simulink library "xps_library"  (Simulink 8.0)
settings: Solver=ode45  SolverMode=SingleTasking  StartTime=0.0  StopTime=10.0  RelTol=1e-3
undefined symbols (not defined in the file): sys_clk, xps_library_software_register_user_data_in
libraries: xbsIndex_r4 x867, simulink x109, dspsigops x81, casper_library_flow_control x68, xps_library x18, casper_library_misc x11
(part 5 of 10)

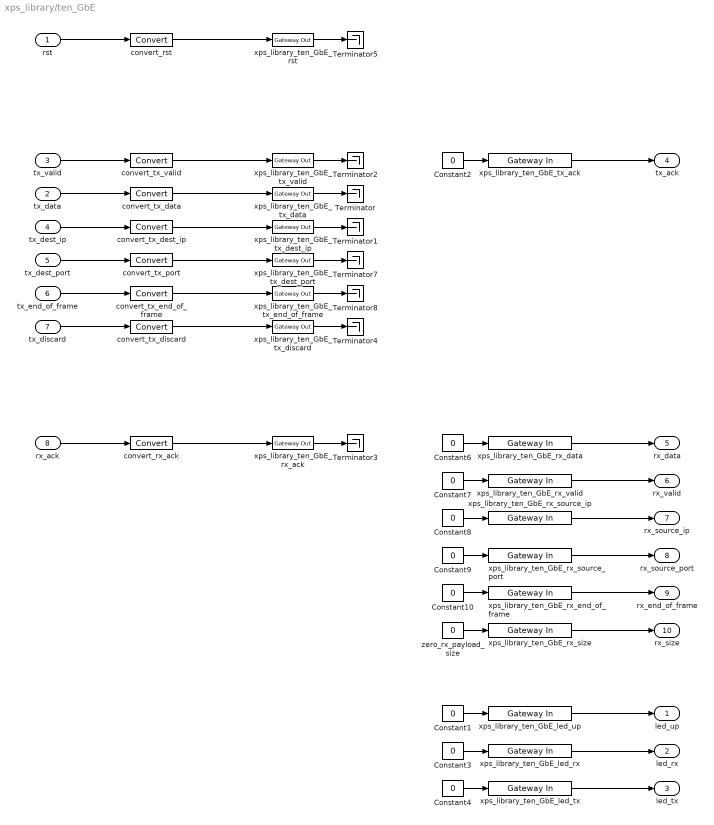
== system xps_library/ten_GbE ==
  rst : Inport
  tx_data : Inport  Port=2
  tx_valid : Inport  Port=3
  tx_dest_ip : Inport  Port=4
  tx_dest_port : Inport  Port=5
  tx_end_of_frame : Inport  Port=6
  tx_discard : Inport  Port=7
  rx_ack : Inport  Port=8
  Constant{1..4,6..10} (9 alike) : Constant  Value=0
  Terminator{,1..5,7..8} (8 alike) : Terminator
  convert_rst : xbsIndex_r4/Convert  gui_display_data_type=Fixed-point  arith_type=Boolean  n_bits=64  bin_pt=0  float_type=Single  exp_bits=8  fraction_bits=24  quantization=Truncate  overflow=Wrap  en=off  latency=0  dbl_ovrd=off  pipeline=off  block_type=convert
      settings: xl_area=[0, 0, 0, 0, 0, 0, 0]
  convert_rx_ack : xbsIndex_r4/Convert  gui_display_data_type=Fixed-point  arith_type=Boolean  n_bits=64  bin_pt=0  float_type=Single  exp_bits=8  fraction_bits=24  quantization=Truncate  overflow=Wrap  en=off  latency=0  dbl_ovrd=off  pipeline=off  block_type=convert
      settings: xl_area=[0, 0, 0, 0, 0, 0, 0]
  convert_tx_data : xbsIndex_r4/Convert  gui_display_data_type=Fixed-point  arith_type=Unsigned  n_bits=64  bin_pt=0  float_type=Single  exp_bits=8  fraction_bits=24  quantization=Truncate  overflow=Wrap  en=off  latency=0  dbl_ovrd=off  pipeline=off  block_type=convert
      settings: xl_area=[0, 0, 0, 0, 0, 0, 0]
  convert_tx_dest_ip : xbsIndex_r4/Convert  gui_display_data_type=Fixed-point  arith_type=Unsigned  n_bits=32  bin_pt=0  float_type=Single  exp_bits=8  fraction_bits=24  quantization=Truncate  overflow=Wrap  en=off  latency=0  dbl_ovrd=off  pipeline=off  block_type=convert
      settings: xl_area=[0, 0, 0, 0, 0, 0, 0]
  convert_tx_discard : xbsIndex_r4/Convert  gui_display_data_type=Fixed-point  arith_type=Boolean  n_bits=1  bin_pt=0  float_type=Single  exp_bits=8  fraction_bits=24  quantization=Truncate  overflow=Wrap  en=off  latency=0  dbl_ovrd=off  pipeline=off  block_type=convert
      settings: xl_area=[0, 0, 0, 0, 0, 0, 0]
  convert_tx_end_of_frame : xbsIndex_r4/Convert  gui_display_data_type=Fixed-point  arith_type=Boolean  n_bits=1  bin_pt=0  float_type=Single  exp_bits=8  fraction_bits=24  quantization=Truncate  overflow=Wrap  en=off  latency=0  dbl_ovrd=off  pipeline=off  block_type=convert
      settings: xl_area=[0, 0, 0, 0, 0, 0, 0]
  convert_tx_port : xbsIndex_r4/Convert  gui_display_data_type=Fixed-point  arith_type=Unsigned  n_bits=16  bin_pt=0  float_type=Single  exp_bits=8  fraction_bits=24  quantization=Truncate  overflow=Wrap  en=off  latency=0  dbl_ovrd=off  pipeline=off  block_type=convert
      settings: xl_area=[0, 0, 0, 0, 0, 0, 0]
  convert_tx_valid : xbsIndex_r4/Convert  gui_display_data_type=Fixed-point  arith_type=Boolean  n_bits=1  bin_pt=0  float_type=Single  exp_bits=8  fraction_bits=24  quantization=Truncate  overflow=Wrap  en=off  latency=0  dbl_ovrd=off  pipeline=off  block_type=convert
      settings: xl_area=[0, 0, 0, 0, 0, 0, 0]
  xps_library_ten_GbE_led_rx : xbsIndex_r4/Gateway In  gui_display_data_type=Fixed-point  arith_type=Boolean  n_bits=1  bin_pt=0  preci_type=Single  exp_width=8  frac_width=24  quantization=Truncate  overflow=Wrap  period=1  dbl_ovrd=off  timing_constraint=None  locs_specified=off  LOCs={}  hdl_port=on  block_type=gatewayin
      settings: infoedit="Gateway in block.  Converts inputs of type Simulink integer, double and fixed point to  Xilinx fixed point type.<P><P>Hardware notes:  In hardware these blocks become top level input ports."  xl_area=[0, 0, 0, 0, 0, 0, 0]
  xps_library_ten_GbE_led_tx : xbsIndex_r4/Gateway In  gui_display_data_type=Fixed-point  arith_type=Boolean  n_bits=1  bin_pt=0  preci_type=Single  exp_width=8  frac_width=24  quantization=Truncate  overflow=Wrap  period=1  dbl_ovrd=off  timing_constraint=None  locs_specified=off  LOCs={}  hdl_port=on  block_type=gatewayin
      settings: infoedit="Gateway in block.  Converts inputs of type Simulink integer, double and fixed point to  Xilinx fixed point type.<P><P>Hardware notes:  In hardware these blocks become top level input ports."  xl_area=[0, 0, 0, 0, 0, 0, 0]
  xps_library_ten_GbE_led_up : xbsIndex_r4/Gateway In  gui_display_data_type=Fixed-point  arith_type=Boolean  n_bits=1  bin_pt=0  preci_type=Single  exp_width=8  frac_width=24  quantization=Truncate  overflow=Wrap  period=1  dbl_ovrd=off  timing_constraint=None  locs_specified=off  LOCs={}  hdl_port=on  block_type=gatewayin
      settings: infoedit="Gateway in block.  Converts inputs of type Simulink integer, double and fixed point to  Xilinx fixed point type.<P><P>Hardware notes:  In hardware these blocks become top level input ports."  xl_area=[0, 0, 0, 0, 0, 0, 0]
  xps_library_ten_GbE_rst : xbsIndex_r4/Gateway Out  hdl_port=on  timing_constraint=None  locs_specified=off  LOCs={}  block_type=gatewayout
      settings: infoedit="Gateway out block.  Converts Xilinx fixed point inputs into ouputs of type Simulink integer, double, or fixed point.<P><P>Hardware notes:  In hardware these blocks become top level output ports or are discarded, depending on how they are configured."  xl_area=[0, 0, 0, 0, 0, 0, 0]
  xps_library_ten_GbE_rx_ack : xbsIndex_r4/Gateway Out  hdl_port=on  timing_constraint=None  locs_specified=off  LOCs={}  block_type=gatewayout
      settings: infoedit="Gateway out block.  Converts Xilinx fixed point inputs into ouputs of type Simulink integer, double, or fixed point.<P><P>Hardware notes:  In hardware these blocks become top level output ports or are discarded, depending on how they are configured."  xl_area=[0, 0, 0, 0, 0, 0, 0]
  xps_library_ten_GbE_rx_data : xbsIndex_r4/Gateway In  gui_display_data_type=Fixed-point  arith_type=Unsigned  n_bits=64  bin_pt=0  preci_type=Single  exp_width=8  frac_width=24  quantization=Truncate  overflow=Wrap  period=1  dbl_ovrd=off  timing_constraint=None  locs_specified=off  LOCs={}  hdl_port=on  block_type=gatewayin
      settings: infoedit="Gateway in block.  Converts inputs of type Simulink integer, double and fixed point to  Xilinx fixed point type.<P><P>Hardware notes:  In hardware these blocks become top level input ports."  xl_area=[0, 0, 0, 0, 0, 0, 0]
  xps_library_ten_GbE_rx_end_of_frame : xbsIndex_r4/Gateway In  gui_display_data_type=Fixed-point  arith_type=Boolean  n_bits=1  bin_pt=0  preci_type=Single  exp_width=8  frac_width=24  quantization=Truncate  overflow=Wrap  period=1  dbl_ovrd=off  timing_constraint=None  locs_specified=off  LOCs={}  hdl_port=on  block_type=gatewayin
      settings: infoedit="Gateway in block.  Converts inputs of type Simulink integer, double and fixed point to  Xilinx fixed point type.<P><P>Hardware notes:  In hardware these blocks become top level input ports."  xl_area=[0, 0, 0, 0, 0, 0, 0]
  xps_library_ten_GbE_rx_size : xbsIndex_r4/Gateway In  gui_display_data_type=Fixed-point  arith_type=Unsigned  n_bits=16  bin_pt=0  preci_type=Single  exp_width=8  frac_width=24  quantization=Truncate  overflow=Wrap  period=1  dbl_ovrd=off  timing_constraint=None  locs_specified=off  LOCs={}  hdl_port=on  block_type=gatewayin
      settings: infoedit="Gateway in block.  Converts inputs of type Simulink integer, double and fixed point to  Xilinx fixed point type.<P><P>Hardware notes:  In hardware these blocks become top level input ports."  xl_area=[0, 0, 0, 0, 0, 0, 0]
  xps_library_ten_GbE_rx_source_ip : xbsIndex_r4/Gateway In  gui_display_data_type=Fixed-point  arith_type=Unsigned  n_bits=32  bin_pt=0  preci_type=Single  exp_width=8  frac_width=24  quantization=Truncate  overflow=Wrap  period=1  dbl_ovrd=off  timing_constraint=None  locs_specified=off  LOCs={}  hdl_port=on  block_type=gatewayin
      settings: infoedit="Gateway in block.  Converts inputs of type Simulink integer, double and fixed point to  Xilinx fixed point type.<P><P>Hardware notes:  In hardware these blocks become top level input ports."  xl_area=[0, 0, 0, 0, 0, 0, 0]
  xps_library_ten_GbE_rx_source_port : xbsIndex_r4/Gateway In  gui_display_data_type=Fixed-point  arith_type=Unsigned  n_bits=16  bin_pt=0  preci_type=Single  exp_width=8  frac_width=24  quantization=Truncate  overflow=Wrap  period=1  dbl_ovrd=off  timing_constraint=None  locs_specified=off  LOCs={}  hdl_port=on  block_type=gatewayin
      settings: infoedit="Gateway in block.  Converts inputs of type Simulink integer, double and fixed point to  Xilinx fixed point type.<P><P>Hardware notes:  In hardware these blocks become top level input ports."  xl_area=[0, 0, 0, 0, 0, 0, 0]
  xps_library_ten_GbE_rx_valid : xbsIndex_r4/Gateway In  gui_display_data_type=Fixed-point  arith_type=Boolean  n_bits=1  bin_pt=0  preci_type=Single  exp_width=8  frac_width=24  quantization=Truncate  overflow=Wrap  period=1  dbl_ovrd=off  timing_constraint=None  locs_specified=off  LOCs={}  hdl_port=on  block_type=gatewayin
      settings: infoedit="Gateway in block.  Converts inputs of type Simulink integer, double and fixed point to  Xilinx fixed point type.<P><P>Hardware notes:  In hardware these blocks become top level input ports."  xl_area=[0, 0, 0, 0, 0, 0, 0]
  xps_library_ten_GbE_tx_ack : xbsIndex_r4/Gateway In  gui_display_data_type=Fixed-point  arith_type=Boolean  n_bits=1  bin_pt=0  preci_type=Single  exp_width=8  frac_width=24  quantization=Truncate  overflow=Wrap  period=1  dbl_ovrd=off  timing_constraint=None  locs_specified=off  LOCs={}  hdl_port=on  block_type=gatewayin
      settings: infoedit="Gateway in block.  Converts inputs of type Simulink integer, double and fixed point to  Xilinx fixed point type.<P><P>Hardware notes:  In hardware these blocks become top level input ports."  xl_area=[0, 0, 0, 0, 0, 0, 0]
  xps_library_ten_GbE_tx_data : xbsIndex_r4/Gateway Out  hdl_port=on  timing_constraint=None  locs_specified=off  LOCs={}  block_type=gatewayout
      settings: infoedit="Gateway out block.  Converts Xilinx fixed point inputs into ouputs of type Simulink integer, double, or fixed point.<P><P>Hardware notes:  In hardware these blocks become top level output ports or are discarded, depending on how they are configured."  xl_area=[0, 0, 0, 0, 0, 0, 0]
  xps_library_ten_GbE_tx_dest_ip : xbsIndex_r4/Gateway Out  hdl_port=on  timing_constraint=None  locs_specified=off  LOCs={}  block_type=gatewayout
      settings: infoedit="Gateway out block.  Converts Xilinx fixed point inputs into ouputs of type Simulink integer, double, or fixed point.<P><P>Hardware notes:  In hardware these blocks become top level output ports or are discarded, depending on how they are configured."  xl_area=[0, 0, 0, 0, 0, 0, 0]
  xps_library_ten_GbE_tx_dest_port : xbsIndex_r4/Gateway Out  hdl_port=on  timing_constraint=None  locs_specified=off  LOCs={}  block_type=gatewayout
      settings: infoedit="Gateway out block.  Converts Xilinx fixed point inputs into ouputs of type Simulink integer, double, or fixed point.<P><P>Hardware notes:  In hardware these blocks become top level output ports or are discarded, depending on how they are configured."  xl_area=[0, 0, 0, 0, 0, 0, 0]
  xps_library_ten_GbE_tx_discard : xbsIndex_r4/Gateway Out  hdl_port=on  timing_constraint=None  locs_specified=off  LOCs={}  block_type=gatewayout
      settings: infoedit="Gateway out block.  Converts Xilinx fixed point inputs into ouputs of type Simulink integer, double, or fixed point.<P><P>Hardware notes:  In hardware these blocks become top level output ports or are discarded, depending on how they are configured."  xl_area=[0, 0, 0, 0, 0, 0, 0]
  xps_library_ten_GbE_tx_end_of_frame : xbsIndex_r4/Gateway Out  hdl_port=on  timing_constraint=None  locs_specified=off  LOCs={}  block_type=gatewayout
      settings: infoedit="Gateway out block.  Converts Xilinx fixed point inputs into ouputs of type Simulink integer, double, or fixed point.<P><P>Hardware notes:  In hardware these blocks become top level output ports or are discarded, depending on how they are configured."  xl_area=[0, 0, 0, 0, 0, 0, 0]
  xps_library_ten_GbE_tx_valid : xbsIndex_r4/Gateway Out  hdl_port=on  timing_constraint=None  locs_specified=off  LOCs={}  block_type=gatewayout
      settings: infoedit="Gateway out block.  Converts Xilinx fixed point inputs into ouputs of type Simulink integer, double, or fixed point.<P><P>Hardware notes:  In hardware these blocks become top level output ports or are discarded, depending on how they are configured."  xl_area=[0, 0, 0, 0, 0, 0, 0]
  zero_rx_payload_size : Constant  Value=0
  led_up : Outport
  led_rx : Outport  Port=2
  led_tx : Outport  Port=3
  tx_ack : Outport  Port=4
  rx_data : Outport  Port=5
  rx_valid : Outport  Port=6
  rx_source_ip : Outport  Port=7
  rx_source_port : Outport  Port=8
  rx_end_of_frame : Outport  Port=9
  rx_size : Outport  Port=10
  wires:
  rx_ack/1 -> convert_rx_ack/1
  convert_rx_ack/1 -> xps_library_ten_GbE_rx_ack/1
  xps_library_ten_GbE_rx_data/1 -> rx_data/1
  tx_data/1 -> convert_tx_data/1
  convert_tx_data/1 -> xps_library_ten_GbE_tx_data/1
  tx_dest_ip/1 -> convert_tx_dest_ip/1
  convert_tx_dest_ip/1 -> xps_library_ten_GbE_tx_dest_ip/1
  tx_valid/1 -> convert_tx_valid/1
  convert_tx_valid/1 -> xps_library_ten_GbE_tx_valid/1
  xps_library_ten_GbE_tx_ack/1 -> tx_ack/1
  xps_library_ten_GbE_tx_data/1 -> Terminator/1
  xps_library_ten_GbE_tx_dest_ip/1 -> Terminator1/1
  xps_library_ten_GbE_tx_valid/1 -> Terminator2/1
  Constant2/1 -> xps_library_ten_GbE_tx_ack/1
  Constant6/1 -> xps_library_ten_GbE_rx_data/1
  xps_library_ten_GbE_rx_ack/1 -> Terminator3/1
  Constant7/1 -> xps_library_ten_GbE_rx_valid/1
  xps_library_ten_GbE_rx_valid/1 -> rx_valid/1
  rst/1 -> convert_rst/1
  convert_rst/1 -> xps_library_ten_GbE_rst/1
  xps_library_ten_GbE_rst/1 -> Terminator5/1
  tx_dest_port/1 -> convert_tx_port/1
  convert_tx_port/1 -> xps_library_ten_GbE_tx_dest_port/1
  xps_library_ten_GbE_tx_dest_port/1 -> Terminator7/1
  tx_end_of_frame/1 -> convert_tx_end_of_frame/1
  convert_tx_end_of_frame/1 -> xps_library_ten_GbE_tx_end_of_frame/1
  xps_library_ten_GbE_tx_end_of_frame/1 -> Terminator8/1
  xps_library_ten_GbE_rx_source_ip/1 -> rx_source_ip/1
  Constant8/1 -> xps_library_ten_GbE_rx_source_ip/1
  Constant9/1 -> xps_library_ten_GbE_rx_source_port/1
  xps_library_ten_GbE_rx_source_port/1 -> rx_source_port/1
  Constant10/1 -> xps_library_ten_GbE_rx_end_of_frame/1
  xps_library_ten_GbE_rx_end_of_frame/1 -> rx_end_of_frame/1
  Constant1/1 -> xps_library_ten_GbE_led_up/1
  xps_library_ten_GbE_led_up/1 -> led_up/1
  Constant3/1 -> xps_library_ten_GbE_led_rx/1
  xps_library_ten_GbE_led_rx/1 -> led_rx/1
  Constant4/1 -> xps_library_ten_GbE_led_tx/1
  xps_library_ten_GbE_led_tx/1 -> led_tx/1
  zero_rx_payload_size/1 -> xps_library_ten_GbE_rx_size/1
  xps_library_ten_GbE_rx_size/1 -> rx_size/1
  tx_discard/1 -> convert_tx_discard/1
  convert_tx_discard/1 -> xps_library_ten_GbE_tx_discard/1
  xps_library_ten_GbE_tx_discard/1 -> Terminator4/1

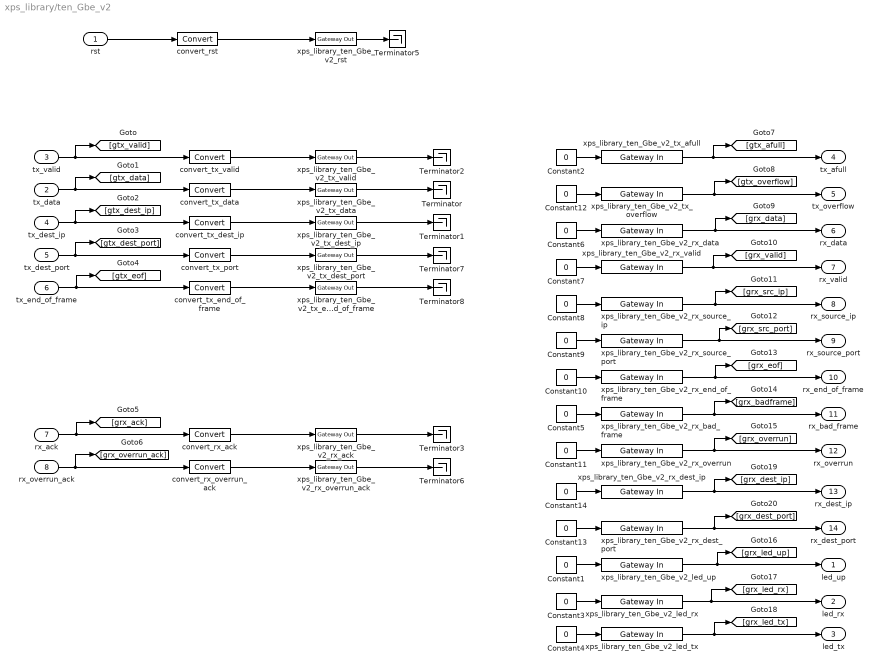
== system xps_library/ten_Gbe_v2 ==
  rst : Inport
  tx_data : Inport  Port=2
  tx_valid : Inport  Port=3
  tx_dest_ip : Inport  Port=4
  tx_dest_port : Inport  Port=5
  tx_end_of_frame : Inport  Port=6
  rx_ack : Inport  Port=7
  rx_overrun_ack : Inport  Port=8
  Constant{1..14} (14 alike) : Constant  Value=0
  Terminator{,1..3,5..8} (8 alike) : Terminator
  convert_rst : xbsIndex_r4/Convert  gui_display_data_type=Fixed-point  arith_type=Boolean  n_bits=64  bin_pt=0  float_type=Single  exp_bits=8  fraction_bits=24  quantization=Truncate  overflow=Wrap  en=off  latency=0  dbl_ovrd=off  pipeline=off  block_type=convert
      settings: xl_area=[0, 0, 0, 0, 0, 0, 0]
  convert_rx_ack : xbsIndex_r4/Convert  gui_display_data_type=Fixed-point  arith_type=Boolean  n_bits=64  bin_pt=0  float_type=Single  exp_bits=8  fraction_bits=24  quantization=Truncate  overflow=Wrap  en=off  latency=0  dbl_ovrd=off  pipeline=off  block_type=convert
      settings: xl_area=[0, 0, 0, 0, 0, 0, 0]
  convert_rx_overrun_ack : xbsIndex_r4/Convert  gui_display_data_type=Fixed-point  arith_type=Boolean  n_bits=64  bin_pt=0  float_type=Single  exp_bits=8  fraction_bits=24  quantization=Truncate  overflow=Wrap  en=off  latency=0  dbl_ovrd=off  pipeline=off  block_type=convert
      settings: xl_area=[0, 0, 0, 0, 0, 0, 0]
  convert_tx_data : xbsIndex_r4/Convert  gui_display_data_type=Fixed-point  arith_type=Unsigned  n_bits=64  bin_pt=0  float_type=Single  exp_bits=8  fraction_bits=24  quantization=Truncate  overflow=Wrap  en=off  latency=0  dbl_ovrd=off  pipeline=off  block_type=convert
      settings: xl_area=[0, 0, 0, 0, 0, 0, 0]
  convert_tx_dest_ip : xbsIndex_r4/Convert  gui_display_data_type=Fixed-point  arith_type=Unsigned  n_bits=32  bin_pt=0  float_type=Single  exp_bits=8  fraction_bits=24  quantization=Truncate  overflow=Wrap  en=off  latency=0  dbl_ovrd=off  pipeline=off  block_type=convert
      settings: xl_area=[0, 0, 0, 0, 0, 0, 0]
  convert_tx_end_of_frame : xbsIndex_r4/Convert  gui_display_data_type=Fixed-point  arith_type=Boolean  n_bits=1  bin_pt=0  float_type=Single  exp_bits=8  fraction_bits=24  quantization=Truncate  overflow=Wrap  en=off  latency=0  dbl_ovrd=off  pipeline=off  block_type=convert
      settings: xl_area=[0, 0, 0, 0, 0, 0, 0]
  convert_tx_port : xbsIndex_r4/Convert  gui_display_data_type=Fixed-point  arith_type=Unsigned  n_bits=16  bin_pt=0  float_type=Single  exp_bits=8  fraction_bits=24  quantization=Truncate  overflow=Wrap  en=off  latency=0  dbl_ovrd=off  pipeline=off  block_type=convert
      settings: xl_area=[0, 0, 0, 0, 0, 0, 0]
  convert_tx_valid : xbsIndex_r4/Convert  gui_display_data_type=Fixed-point  arith_type=Boolean  n_bits=1  bin_pt=0  float_type=Single  exp_bits=8  fraction_bits=24  quantization=Truncate  overflow=Wrap  en=off  latency=0  dbl_ovrd=off  pipeline=off  block_type=convert
      settings: xl_area=[0, 0, 0, 0, 0, 0, 0]
  xps_library_ten_Gbe_v2_led_rx : xbsIndex_r4/Gateway In  gui_display_data_type=Fixed-point  arith_type=Boolean  n_bits=1  bin_pt=0  preci_type=Single  exp_width=8  frac_width=24  quantization=Truncate  overflow=Wrap  period=1  dbl_ovrd=off  timing_constraint=None  locs_specified=off  LOCs={}  UseAsADC=off  ADCChannel='1'  inherit_from_input=off  hdl_port=on  block_type=gatewayin
      settings: infoedit="Gateway in block.  Converts inputs of type Simulink integer, double and fixed point to  Xilinx fixed point type.<P><P>Hardware notes:  In hardware these blocks become top level input ports."  xl_area=[0, 0, 0, 0, 0, 0, 0]
  xps_library_ten_Gbe_v2_led_tx : xbsIndex_r4/Gateway In  gui_display_data_type=Fixed-point  arith_type=Boolean  n_bits=1  bin_pt=0  preci_type=Single  exp_width=8  frac_width=24  quantization=Truncate  overflow=Wrap  period=1  dbl_ovrd=off  timing_constraint=None  locs_specified=off  LOCs={}  UseAsADC=off  ADCChannel='1'  inherit_from_input=off  hdl_port=on  block_type=gatewayin
      settings: infoedit="Gateway in block.  Converts inputs of type Simulink integer, double and fixed point to  Xilinx fixed point type.<P><P>Hardware notes:  In hardware these blocks become top level input ports."  xl_area=[0, 0, 0, 0, 0, 0, 0]
  xps_library_ten_Gbe_v2_led_up : xbsIndex_r4/Gateway In  gui_display_data_type=Fixed-point  arith_type=Boolean  n_bits=1  bin_pt=0  preci_type=Single  exp_width=8  frac_width=24  quantization=Truncate  overflow=Wrap  period=1  dbl_ovrd=off  timing_constraint=None  locs_specified=off  LOCs={}  UseAsADC=off  ADCChannel='1'  inherit_from_input=off  hdl_port=on  block_type=gatewayin
      settings: infoedit="Gateway in block.  Converts inputs of type Simulink integer, double and fixed point to  Xilinx fixed point type.<P><P>Hardware notes:  In hardware these blocks become top level input ports."  xl_area=[0, 0, 0, 0, 0, 0, 0]
  xps_library_ten_Gbe_v2_rst : xbsIndex_r4/Gateway Out  inherit_from_input=off  hdl_port=on  timing_constraint=None  locs_specified=off  LOCs={}  UseAsDAC=off  DACChannel='1'  block_type=gatewayout
      settings: infoedit="Gateway out block.  Converts Xilinx fixed point inputs into ouputs of type Simulink integer, double, or fixed point.<P><P>Hardware notes:  In hardware these blocks become top level output ports or are discarded, depending on how they are configured."  xl_area=[0, 0, 0, 0, 0, 0, 0]
  xps_library_ten_Gbe_v2_rx_ack : xbsIndex_r4/Gateway Out  inherit_from_input=off  hdl_port=on  timing_constraint=None  locs_specified=off  LOCs={}  UseAsDAC=off  DACChannel='1'  block_type=gatewayout
      settings: infoedit="Gateway out block.  Converts Xilinx fixed point inputs into ouputs of type Simulink integer, double, or fixed point.<P><P>Hardware notes:  In hardware these blocks become top level output ports or are discarded, depending on how they are configured."  xl_area=[0, 0, 0, 0, 0, 0, 0]
  xps_library_ten_Gbe_v2_rx_bad_frame : xbsIndex_r4/Gateway In  gui_display_data_type=Fixed-point  arith_type=Boolean  n_bits=1  bin_pt=0  preci_type=Single  exp_width=8  frac_width=24  quantization=Truncate  overflow=Wrap  period=1  dbl_ovrd=off  timing_constraint=None  locs_specified=off  LOCs={}  UseAsADC=off  ADCChannel='1'  inherit_from_input=off  hdl_port=on  block_type=gatewayin
      settings: infoedit="Gateway in block.  Converts inputs of type Simulink integer, double and fixed point to  Xilinx fixed point type.<P><P>Hardware notes:  In hardware these blocks become top level input ports."  xl_area=[0, 0, 0, 0, 0, 0, 0]
  xps_library_ten_Gbe_v2_rx_data : xbsIndex_r4/Gateway In  gui_display_data_type=Fixed-point  arith_type=Unsigned  n_bits=64  bin_pt=0  preci_type=Single  exp_width=8  frac_width=24  quantization=Truncate  overflow=Wrap  period=1  dbl_ovrd=off  timing_constraint=None  locs_specified=off  LOCs={}  UseAsADC=off  ADCChannel='1'  inherit_from_input=off  hdl_port=on  block_type=gatewayin
      settings: infoedit="Gateway in block.  Converts inputs of type Simulink integer, double and fixed point to  Xilinx fixed point type.<P><P>Hardware notes:  In hardware these blocks become top level input ports."  xl_area=[0, 0, 0, 0, 0, 0, 0]
  xps_library_ten_Gbe_v2_rx_dest_ip : xbsIndex_r4/Gateway In  gui_display_data_type=Fixed-point  arith_type=Unsigned  n_bits=32  bin_pt=0  preci_type=Single  exp_width=8  frac_width=24  quantization=Truncate  overflow=Wrap  period=1  dbl_ovrd=off  timing_constraint=None  locs_specified=off  LOCs={}  UseAsADC=off  ADCChannel='1'  inherit_from_input=off  hdl_port=on  block_type=gatewayin
      settings: xl_area=[0, 0, 0, 0, 0, 0, 0]
  xps_library_ten_Gbe_v2_rx_dest_port : xbsIndex_r4/Gateway In  gui_display_data_type=Fixed-point  arith_type=Unsigned  n_bits=16  bin_pt=0  preci_type=Single  exp_width=8  frac_width=24  quantization=Truncate  overflow=Wrap  period=1  dbl_ovrd=off  timing_constraint=None  locs_specified=off  LOCs={}  UseAsADC=off  ADCChannel='1'  inherit_from_input=off  hdl_port=on  block_type=gatewayin
      settings: xl_area=[0, 0, 0, 0, 0, 0, 0]
  xps_library_ten_Gbe_v2_rx_end_of_frame : xbsIndex_r4/Gateway In  gui_display_data_type=Fixed-point  arith_type=Boolean  n_bits=1  bin_pt=0  preci_type=Single  exp_width=8  frac_width=24  quantization=Truncate  overflow=Wrap  period=1  dbl_ovrd=off  timing_constraint=None  locs_specified=off  LOCs={}  UseAsADC=off  ADCChannel='1'  inherit_from_input=off  hdl_port=on  block_type=gatewayin
      settings: infoedit="Gateway in block.  Converts inputs of type Simulink integer, double and fixed point to  Xilinx fixed point type.<P><P>Hardware notes:  In hardware these blocks become top level input ports."  xl_area=[0, 0, 0, 0, 0, 0, 0]
  xps_library_ten_Gbe_v2_rx_overrun : xbsIndex_r4/Gateway In  gui_display_data_type=Fixed-point  arith_type=Boolean  n_bits=1  bin_pt=0  preci_type=Single  exp_width=8  frac_width=24  quantization=Truncate  overflow=Wrap  period=1  dbl_ovrd=off  timing_constraint=None  locs_specified=off  LOCs={}  UseAsADC=off  ADCChannel='1'  inherit_from_input=off  hdl_port=on  block_type=gatewayin
      settings: infoedit="Gateway in block.  Converts inputs of type Simulink integer, double and fixed point to  Xilinx fixed point type.<P><P>Hardware notes:  In hardware these blocks become top level input ports."  xl_area=[0, 0, 0, 0, 0, 0, 0]
  xps_library_ten_Gbe_v2_rx_overrun_ack : xbsIndex_r4/Gateway Out  inherit_from_input=off  hdl_port=on  timing_constraint=None  locs_specified=off  LOCs={}  UseAsDAC=off  DACChannel='1'  block_type=gatewayout
      settings: infoedit="Gateway out block.  Converts Xilinx fixed point inputs into ouputs of type Simulink integer, double, or fixed point.<P><P>Hardware notes:  In hardware these blocks become top level output ports or are discarded, depending on how they are configured."  xl_area=[0, 0, 0, 0, 0, 0, 0]
  xps_library_ten_Gbe_v2_rx_source_ip : xbsIndex_r4/Gateway In  gui_display_data_type=Fixed-point  arith_type=Unsigned  n_bits=32  bin_pt=0  preci_type=Single  exp_width=8  frac_width=24  quantization=Truncate  overflow=Wrap  period=1  dbl_ovrd=off  timing_constraint=None  locs_specified=off  LOCs={}  UseAsADC=off  ADCChannel='1'  inherit_from_input=off  hdl_port=on  block_type=gatewayin
      settings: infoedit="Gateway in block.  Converts inputs of type Simulink integer, double and fixed point to  Xilinx fixed point type.<P><P>Hardware notes:  In hardware these blocks become top level input ports."  xl_area=[0, 0, 0, 0, 0, 0, 0]
  xps_library_ten_Gbe_v2_rx_source_port : xbsIndex_r4/Gateway In  gui_display_data_type=Fixed-point  arith_type=Unsigned  n_bits=16  bin_pt=0  preci_type=Single  exp_width=8  frac_width=24  quantization=Truncate  overflow=Wrap  period=1  dbl_ovrd=off  timing_constraint=None  locs_specified=off  LOCs={}  UseAsADC=off  ADCChannel='1'  inherit_from_input=off  hdl_port=on  block_type=gatewayin
      settings: infoedit="Gateway in block.  Converts inputs of type Simulink integer, double and fixed point to  Xilinx fixed point type.<P><P>Hardware notes:  In hardware these blocks become top level input ports."  xl_area=[0, 0, 0, 0, 0, 0, 0]
  xps_library_ten_Gbe_v2_rx_valid : xbsIndex_r4/Gateway In  gui_display_data_type=Fixed-point  arith_type=Boolean  n_bits=1  bin_pt=0  preci_type=Single  exp_width=8  frac_width=24  quantization=Truncate  overflow=Wrap  period=1  dbl_ovrd=off  timing_constraint=None  locs_specified=off  LOCs={}  UseAsADC=off  ADCChannel='1'  inherit_from_input=off  hdl_port=on  block_type=gatewayin
      settings: infoedit="Gateway in block.  Converts inputs of type Simulink integer, double and fixed point to  Xilinx fixed point type.<P><P>Hardware notes:  In hardware these blocks become top level input ports."  xl_area=[0, 0, 0, 0, 0, 0, 0]
  xps_library_ten_Gbe_v2_tx_afull : xbsIndex_r4/Gateway In  gui_display_data_type=Fixed-point  arith_type=Boolean  n_bits=1  bin_pt=0  preci_type=Single  exp_width=8  frac_width=24  quantization=Truncate  overflow=Wrap  period=1  dbl_ovrd=off  timing_constraint=None  locs_specified=off  LOCs={}  UseAsADC=off  ADCChannel='1'  inherit_from_input=off  hdl_port=on  block_type=gatewayin
      settings: infoedit="Gateway in block.  Converts inputs of type Simulink integer, double and fixed point to  Xilinx fixed point type.<P><P>Hardware notes:  In hardware these blocks become top level input ports."  xl_area=[0, 0, 0, 0, 0, 0, 0]
  xps_library_ten_Gbe_v2_tx_data : xbsIndex_r4/Gateway Out  inherit_from_input=off  hdl_port=on  timing_constraint=None  locs_specified=off  LOCs={}  UseAsDAC=off  DACChannel='1'  block_type=gatewayout
      settings: infoedit="Gateway out block.  Converts Xilinx fixed point inputs into ouputs of type Simulink integer, double, or fixed point.<P><P>Hardware notes:  In hardware these blocks become top level output ports or are discarded, depending on how they are configured."  xl_area=[0, 0, 0, 0, 0, 0, 0]
  xps_library_ten_Gbe_v2_tx_dest_ip : xbsIndex_r4/Gateway Out  inherit_from_input=off  hdl_port=on  timing_constraint=None  locs_specified=off  LOCs={}  UseAsDAC=off  DACChannel='1'  block_type=gatewayout
      settings: infoedit="Gateway out block.  Converts Xilinx fixed point inputs into ouputs of type Simulink integer, double, or fixed point.<P><P>Hardware notes:  In hardware these blocks become top level output ports or are discarded, depending on how they are configured."  xl_area=[0, 0, 0, 0, 0, 0, 0]
  xps_library_ten_Gbe_v2_tx_dest_port : xbsIndex_r4/Gateway Out  inherit_from_input=off  hdl_port=on  timing_constraint=None  locs_specified=off  LOCs={}  UseAsDAC=off  DACChannel='1'  block_type=gatewayout
      settings: infoedit="Gateway out block.  Converts Xilinx fixed point inputs into ouputs of type Simulink integer, double, or fixed point.<P><P>Hardware notes:  In hardware these blocks become top level output ports or are discarded, depending on how they are configured."  xl_area=[0, 0, 0, 0, 0, 0, 0]
  xps_library_ten_Gbe_v2_tx_end_of_frame : xbsIndex_r4/Gateway Out  inherit_from_input=off  hdl_port=on  timing_constraint=None  locs_specified=off  LOCs={}  UseAsDAC=off  DACChannel='1'  block_type=gatewayout
      settings: infoedit="Gateway out block.  Converts Xilinx fixed point inputs into ouputs of type Simulink integer, double, or fixed point.<P><P>Hardware notes:  In hardware these blocks become top level output ports or are discarded, depending on how they are configured."  xl_area=[0, 0, 0, 0, 0, 0, 0]
  xps_library_ten_Gbe_v2_tx_overflow : xbsIndex_r4/Gateway In  gui_display_data_type=Fixed-point  arith_type=Boolean  n_bits=1  bin_pt=0  preci_type=Single  exp_width=8  frac_width=24  quantization=Truncate  overflow=Wrap  period=1  dbl_ovrd=off  timing_constraint=None  locs_specified=off  LOCs={}  UseAsADC=off  ADCChannel='1'  inherit_from_input=off  hdl_port=on  block_type=gatewayin
      settings: infoedit="Gateway in block.  Converts inputs of type Simulink integer, double and fixed point to  Xilinx fixed point type.<P><P>Hardware notes:  In hardware these blocks become top level input ports."  xl_area=[0, 0, 0, 0, 0, 0, 0]
  xps_library_ten_Gbe_v2_tx_valid : xbsIndex_r4/Gateway Out  inherit_from_input=off  hdl_port=on  timing_constraint=None  locs_specified=off  LOCs={}  UseAsDAC=off  DACChannel='1'  block_type=gatewayout
      settings: infoedit="Gateway out block.  Converts Xilinx fixed point inputs into ouputs of type Simulink integer, double, or fixed point.<P><P>Hardware notes:  In hardware these blocks become top level output ports or are discarded, depending on how they are configured."  xl_area=[0, 0, 0, 0, 0, 0, 0]
  led_up : Outport
  led_rx : Outport  Port=2
  led_tx : Outport  Port=3
  tx_afull : Outport  Port=4
  tx_overflow : Outport  Port=5
  rx_data : Outport  Port=6
  rx_valid : Outport  Port=7
  rx_source_ip : Outport  Port=8
  rx_source_port : Outport  Port=9
  rx_end_of_frame : Outport  Port=10
  rx_bad_frame : Outport  Port=11
  rx_overrun : Outport  Port=12
  rx_dest_ip : Outport  Port=13
  rx_dest_port : Outport  Port=14
  wires:
  xps_library_ten_Gbe_v2_tx_overflow/1 -> [gtx_overflow], tx_overflow/1
  Constant12/1 -> xps_library_ten_Gbe_v2_tx_overflow/1
  rx_overrun_ack/1 -> [grx_overrun_ack], convert_rx_overrun_ack/1
  convert_rx_overrun_ack/1 -> xps_library_ten_Gbe_v2_rx_overrun_ack/1
  xps_library_ten_Gbe_v2_rx_overrun_ack/1 -> Terminator6/1
  Constant11/1 -> xps_library_ten_Gbe_v2_rx_overrun/1
  xps_library_ten_Gbe_v2_rx_overrun/1 -> [grx_overrun], rx_overrun/1
  Constant5/1 -> xps_library_ten_Gbe_v2_rx_bad_frame/1
  xps_library_ten_Gbe_v2_rx_bad_frame/1 -> [grx_badframe], rx_bad_frame/1
  rx_ack/1 -> [grx_ack], convert_rx_ack/1
  convert_rx_ack/1 -> xps_library_ten_Gbe_v2_rx_ack/1
  xps_library_ten_Gbe_v2_rx_data/1 -> [grx_data], rx_data/1
  tx_data/1 -> [gtx_data], convert_tx_data/1
  convert_tx_data/1 -> xps_library_ten_Gbe_v2_tx_data/1
  tx_dest_ip/1 -> [gtx_dest_ip], convert_tx_dest_ip/1
  convert_tx_dest_ip/1 -> xps_library_ten_Gbe_v2_tx_dest_ip/1
  tx_valid/1 -> [gtx_valid], convert_tx_valid/1
  convert_tx_valid/1 -> xps_library_ten_Gbe_v2_tx_valid/1
  xps_library_ten_Gbe_v2_tx_afull/1 -> [gtx_afull], tx_afull/1
  xps_library_ten_Gbe_v2_tx_data/1 -> Terminator/1
  xps_library_ten_Gbe_v2_tx_dest_ip/1 -> Terminator1/1
  xps_library_ten_Gbe_v2_tx_valid/1 -> Terminator2/1
  Constant2/1 -> xps_library_ten_Gbe_v2_tx_afull/1
  Constant6/1 -> xps_library_ten_Gbe_v2_rx_data/1
  xps_library_ten_Gbe_v2_rx_ack/1 -> Terminator3/1
  Constant7/1 -> xps_library_ten_Gbe_v2_rx_valid/1
  xps_library_ten_Gbe_v2_rx_valid/1 -> [grx_valid], rx_valid/1
  rst/1 -> convert_rst/1
  convert_rst/1 -> xps_library_ten_Gbe_v2_rst/1
  xps_library_ten_Gbe_v2_rst/1 -> Terminator5/1
  tx_dest_port/1 -> [gtx_dest_port], convert_tx_port/1
  convert_tx_port/1 -> xps_library_ten_Gbe_v2_tx_dest_port/1
  xps_library_ten_Gbe_v2_tx_dest_port/1 -> Terminator7/1
  tx_end_of_frame/1 -> [gtx_eof], convert_tx_end_of_frame/1
  convert_tx_end_of_frame/1 -> xps_library_ten_Gbe_v2_tx_end_of_frame/1
  xps_library_ten_Gbe_v2_tx_end_of_frame/1 -> Terminator8/1
  xps_library_ten_Gbe_v2_rx_source_ip/1 -> [grx_src_ip], rx_source_ip/1
  Constant8/1 -> xps_library_ten_Gbe_v2_rx_source_ip/1
  Constant9/1 -> xps_library_ten_Gbe_v2_rx_source_port/1
  xps_library_ten_Gbe_v2_rx_source_port/1 -> [grx_src_port], rx_source_port/1
  Constant10/1 -> xps_library_ten_Gbe_v2_rx_end_of_frame/1
  xps_library_ten_Gbe_v2_rx_end_of_frame/1 -> [grx_eof], rx_end_of_frame/1
  Constant1/1 -> xps_library_ten_Gbe_v2_led_up/1
  xps_library_ten_Gbe_v2_led_up/1 -> [grx_led_up], led_up/1
  Constant3/1 -> xps_library_ten_Gbe_v2_led_rx/1
  xps_library_ten_Gbe_v2_led_rx/1 -> [grx_led_rx], led_rx/1
  Constant4/1 -> xps_library_ten_Gbe_v2_led_tx/1
  xps_library_ten_Gbe_v2_led_tx/1 -> [grx_led_tx], led_tx/1
  Constant13/1 -> xps_library_ten_Gbe_v2_rx_dest_port/1
  xps_library_ten_Gbe_v2_rx_dest_port/1 -> rx_dest_port/1, [grx_dest_port]
  Constant14/1 -> xps_library_ten_Gbe_v2_rx_dest_ip/1
  xps_library_ten_Gbe_v2_rx_dest_ip/1 -> rx_dest_ip/1, [grx_dest_ip]

== system xps_library/ADCs/adc083000_ctrl ==
  conf : Inport
  sdata_bus : Inport  Port=2
  Convert : xbsIndex_r4/Convert  gui_display_data_type=Fixed-point  arith_type=Unsigned  n_bits=3  bin_pt=0  float_type=Single  exp_bits=8  fraction_bits=24  quantization=Truncate  overflow=Wrap  en=off  latency=2  dbl_ovrd=off  pipeline=off  block_type=convert
      settings: block_version=11.4
  Convert1 : xbsIndex_r4/Convert  gui_display_data_type=Fixed-point  arith_type=Unsigned  n_bits=32  bin_pt=0  float_type=Single  exp_bits=8  fraction_bits=24  quantization=Truncate  overflow=Wrap  en=off  latency=2  dbl_ovrd=off  pipeline=off  block_type=convert
      settings: block_version=11.4
  Slice : xbsIndex_r4/Slice  nbits=3  boolean_output=off  mode=Lower Bit Location + Width  bit1=0  base1=MSB of Input  bit0=0  base0=LSB of Input  dbl_ovrd=off  block_type=slice
  Terminator : Terminator
  Terminator1 : Terminator
  xps_library_ADCs_adc083000_ctrl_conf : xbsIndex_r4/Gateway Out  inherit_from_input=off  hdl_port=on  timing_constraint=None  locs_specified=off  LOCs={}  UseAsDAC=off  DACChannel='1'  block_type=gatewayout
      settings: infoedit="Gateway out block.  Converts Xilinx fixed point inputs into ouputs of type Simulink integer, double, or fixed point.<br><br>Hardware notes:  In hardware these blocks become top level output ports or are discarded, depending on how they are configured."  block_version=11.4
  xps_library_ADCs_adc083000_ctrl_sdata_bus : xbsIndex_r4/Gateway Out  inherit_from_input=off  hdl_port=on  timing_constraint=None  locs_specified=off  LOCs={}  UseAsDAC=off  DACChannel='1'  block_type=gatewayout
      settings: infoedit="Gateway out block.  Converts Xilinx fixed point inputs into ouputs of type Simulink integer, double, or fixed point.<br><br>Hardware notes:  In hardware these blocks become top level output ports or are discarded, depending on how they are configured."  block_version=11.4
  wires:
  xps_library_ADCs_adc083000_ctrl_sdata_bus/1 -> Terminator1/1
  xps_library_ADCs_adc083000_ctrl_conf/1 -> Terminator/1
  Convert1/1 -> xps_library_ADCs_adc083000_ctrl_sdata_bus/1
  Slice/1 -> Convert/1
  conf/1 -> Slice/1
  Convert/1 -> xps_library_ADCs_adc083000_ctrl_conf/1
  sdata_bus/1 -> Convert1/1

== system xps_library/ADCs/adc16x250-8 ==
  a1_sim : Inport
  a2_sim : Inport  Port=2
  a3_sim : Inport  Port=3
  a4_sim : Inport  Port=4
  b1_sim : Inport  Port=5
  b2_sim : Inport  Port=6
  b3_sim : Inport  Port=7
  b4_sim : Inport  Port=8
  c1_sim : Inport  Port=9
  c2_sim : Inport  Port=10
  c3_sim : Inport  Port=11
  c4_sim : Inport  Port=12
  d1_sim : Inport  Port=13
  d2_sim : Inport  Port=14
  d3_sim : Inport  Port=15
  d4_sim : Inport  Port=16
  xps_library_ADCs_adc16x250_8_a{1..4} (4 alike) : xbsIndex_r4/Gateway In  gui_display_data_type=Fixed-point  arith_type="Signed  (2's comp)"  n_bits=8  bin_pt=7  preci_type=Single  exp_width=8  frac_width=24  quantization="Round  (unbiased: +/- Inf)"  overflow=Saturate  period=1  dbl_ovrd=off  timing_constraint=None  locs_specified=off  LOCs={}  UseAsADC=off  ADCChannel='1'  inherit_from_input=off  hdl_port=on  block_type=gatewayin
  xps_library_ADCs_adc16x250_8_b{1..4} (4 alike) : xbsIndex_r4/Gateway In  gui_display_data_type=Fixed-point  arith_type="Signed  (2's comp)"  n_bits=8  bin_pt=7  preci_type=Single  exp_width=8  frac_width=24  quantization="Round  (unbiased: +/- Inf)"  overflow=Saturate  period=1  dbl_ovrd=off  timing_constraint=None  locs_specified=off  LOCs={}  UseAsADC=off  ADCChannel='1'  inherit_from_input=off  hdl_port=on  block_type=gatewayin
  xps_library_ADCs_adc16x250_8_c{1..4} (4 alike) : xbsIndex_r4/Gateway In  gui_display_data_type=Fixed-point  arith_type="Signed  (2's comp)"  n_bits=8  bin_pt=7  preci_type=Single  exp_width=8  frac_width=24  quantization="Round  (unbiased: +/- Inf)"  overflow=Saturate  period=1  dbl_ovrd=off  timing_constraint=None  locs_specified=off  LOCs={}  UseAsADC=off  ADCChannel='1'  inherit_from_input=off  hdl_port=on  block_type=gatewayin
  xps_library_ADCs_adc16x250_8_d{1..4} (4 alike) : xbsIndex_r4/Gateway In  gui_display_data_type=Fixed-point  arith_type="Signed  (2's comp)"  n_bits=8  bin_pt=7  preci_type=Single  exp_width=8  frac_width=24  quantization="Round  (unbiased: +/- Inf)"  overflow=Saturate  period=1  dbl_ovrd=off  timing_constraint=None  locs_specified=off  LOCs={}  UseAsADC=off  ADCChannel='1'  inherit_from_input=off  hdl_port=on  block_type=gatewayin
  a1 : Outport
  a2 : Outport  Port=2
  a3 : Outport  Port=3
  a4 : Outport  Port=4
  b1 : Outport  Port=5
  b2 : Outport  Port=6
  b3 : Outport  Port=7
  b4 : Outport  Port=8
  c1 : Outport  Port=9
  c2 : Outport  Port=10
  c3 : Outport  Port=11
  c4 : Outport  Port=12
  d1 : Outport  Port=13
  d2 : Outport  Port=14
  d3 : Outport  Port=15
  d4 : Outport  Port=16
  wires:
  a1_sim/1 -> xps_library_ADCs_adc16x250_8_a1/1
  xps_library_ADCs_adc16x250_8_a1/1 -> a1/1  "a1"
  a2_sim/1 -> xps_library_ADCs_adc16x250_8_a2/1
  xps_library_ADCs_adc16x250_8_a2/1 -> a2/1  "a2"
  a3_sim/1 -> xps_library_ADCs_adc16x250_8_a3/1
  xps_library_ADCs_adc16x250_8_a3/1 -> a3/1  "a3"
  a4_sim/1 -> xps_library_ADCs_adc16x250_8_a4/1
  xps_library_ADCs_adc16x250_8_a4/1 -> a4/1  "a4"
  b1_sim/1 -> xps_library_ADCs_adc16x250_8_b1/1
  xps_library_ADCs_adc16x250_8_b1/1 -> b1/1  "b1"
  b2_sim/1 -> xps_library_ADCs_adc16x250_8_b2/1
  xps_library_ADCs_adc16x250_8_b2/1 -> b2/1  "b2"
  b3_sim/1 -> xps_library_ADCs_adc16x250_8_b3/1
  xps_library_ADCs_adc16x250_8_b3/1 -> b3/1  "b3"
  b4_sim/1 -> xps_library_ADCs_adc16x250_8_b4/1
  xps_library_ADCs_adc16x250_8_b4/1 -> b4/1  "b4"
  c1_sim/1 -> xps_library_ADCs_adc16x250_8_c1/1
  xps_library_ADCs_adc16x250_8_c1/1 -> c1/1  "c1"
  c2_sim/1 -> xps_library_ADCs_adc16x250_8_c2/1
  xps_library_ADCs_adc16x250_8_c2/1 -> c2/1  "c2"
  c3_sim/1 -> xps_library_ADCs_adc16x250_8_c3/1
  xps_library_ADCs_adc16x250_8_c3/1 -> c3/1  "c3"
  c4_sim/1 -> xps_library_ADCs_adc16x250_8_c4/1
  xps_library_ADCs_adc16x250_8_c4/1 -> c4/1  "c4"
  d1_sim/1 -> xps_library_ADCs_adc16x250_8_d1/1
  xps_library_ADCs_adc16x250_8_d1/1 -> d1/1  "d1"
  d2_sim/1 -> xps_library_ADCs_adc16x250_8_d2/1
  xps_library_ADCs_adc16x250_8_d2/1 -> d2/1  "d2"
  d3_sim/1 -> xps_library_ADCs_adc16x250_8_d3/1
  xps_library_ADCs_adc16x250_8_d3/1 -> d3/1  "d3"
  d4_sim/1 -> xps_library_ADCs_adc16x250_8_d4/1
  xps_library_ADCs_adc16x250_8_d4/1 -> d4/1  "d4"

== system xps_library/ADCs/adc2x14_400 ==
  adc_snap_test_zdock0_adc2x14_400_user_data_i0 : xbsIndex_r4/Gateway In  gui_display_data_type=Fixed-point  arith_type=Unsigned  n_bits=14  bin_pt=0  preci_type=Single  exp_width=8  frac_width=24  quantization=Truncate  overflow=Wrap  period=1  dbl_ovrd=off  timing_constraint=None  locs_specified=off  LOCs={}  hdl_port=on  block_type=gatewayin
      settings: infoedit="Gateway in block.  Converts inputs of type Simulink integer, double and fixed point to  Xilinx fixed point type.<P><P>Hardware notes:  In hardware these blocks become top level input ports."  xl_area=[0, 0, 0, 0, 0, 0, 0]  block_version=10.1.3
  adc_snap_test_zdock0_adc2x14_400_user_data_i1 : xbsIndex_r4/Gateway In  gui_display_data_type=Fixed-point  arith_type=Unsigned  n_bits=14  bin_pt=0  preci_type=Single  exp_width=8  frac_width=24  quantization=Truncate  overflow=Wrap  period=1  dbl_ovrd=off  timing_constraint=None  locs_specified=off  LOCs={}  hdl_port=on  block_type=gatewayin
      settings: infoedit="Gateway in block.  Converts inputs of type Simulink integer, double and fixed point to  Xilinx fixed point type.<P><P>Hardware notes:  In hardware these blocks become top level input ports."  xl_area=[0, 0, 0, 0, 0, 0, 0]  block_version=10.1.3
  adc_snap_test_zdock0_adc2x14_400_user_data_q0 : xbsIndex_r4/Gateway In  gui_display_data_type=Fixed-point  arith_type=Unsigned  n_bits=14  bin_pt=0  preci_type=Single  exp_width=8  frac_width=24  quantization=Truncate  overflow=Wrap  period=1  dbl_ovrd=off  timing_constraint=None  locs_specified=off  LOCs={}  hdl_port=on  block_type=gatewayin
      settings: infoedit="Gateway in block.  Converts inputs of type Simulink integer, double and fixed point to  Xilinx fixed point type.<P><P>Hardware notes:  In hardware these blocks become top level input ports."  xl_area=[0, 0, 0, 0, 0, 0, 0]  block_version=10.1.3
  adc_snap_test_zdock0_adc2x14_400_user_data_q1 : xbsIndex_r4/Gateway In  gui_display_data_type=Fixed-point  arith_type=Unsigned  n_bits=14  bin_pt=0  preci_type=Single  exp_width=8  frac_width=24  quantization=Truncate  overflow=Wrap  period=1  dbl_ovrd=off  timing_constraint=None  locs_specified=off  LOCs={}  hdl_port=on  block_type=gatewayin
      settings: infoedit="Gateway in block.  Converts inputs of type Simulink integer, double and fixed point to  Xilinx fixed point type.<P><P>Hardware notes:  In hardware these blocks become top level input ports."  xl_area=[0, 0, 0, 0, 0, 0, 0]  block_version=10.1.3
  adc_snap_test_zdock0_adc2x14_400_user_sync : xbsIndex_r4/Gateway In  gui_display_data_type=Fixed-point  arith_type=Boolean  n_bits=1  bin_pt=0  preci_type=Single  exp_width=8  frac_width=24  quantization=Truncate  overflow=Wrap  period=1  dbl_ovrd=off  timing_constraint=None  locs_specified=off  LOCs={}  hdl_port=on  block_type=gatewayin
      settings: infoedit="Gateway in block.  Converts inputs of type Simulink integer, double and fixed point to  Xilinx fixed point type.<P><P>Hardware notes:  In hardware these blocks become top level input ports."  xl_area=[0, 0, 0, 0, 0, 0, 0]  block_version=10.1.3
  conv : Subsystem
      mask help:
      | Converts an (12-bit) unsigned number to 2's complement.
      | This block should eventually be able to handle arbitrary
      | width inputs.
  conv1 : Subsystem
      mask help:
      | Converts an (12-bit) unsigned number to 2's complement.
      | This block should eventually be able to handle arbitrary
      | width inputs.
  conv2 : Subsystem
      mask help:
      | Converts an (12-bit) unsigned number to 2's complement.
      | This block should eventually be able to handle arbitrary
      | width inputs.
  conv3 : Subsystem
      mask help:
      | Converts an (12-bit) unsigned number to 2's complement.
      | This block should eventually be able to handle arbitrary
      | width inputs.
  data_i0 : Outport
  data_i1 : Outport  Port=2
  data_q0 : Outport  Port=3
  data_q1 : Outport  Port=4
  sync : Outport  Port=5
  wires:
  adc_snap_test_zdock0_adc2x14_400_user_sync/1 -> sync/1
  adc_snap_test_zdock0_adc2x14_400_user_data_i0/1 -> conv/1(In1)
  conv/1(Out1) -> data_i0/1
  adc_snap_test_zdock0_adc2x14_400_user_data_q0/1 -> conv2/1(In1)
  conv2/1(Out1) -> data_q0/1
  adc_snap_test_zdock0_adc2x14_400_user_data_i1/1 -> conv1/1(In1)
  conv1/1(Out1) -> data_i1/1
  adc_snap_test_zdock0_adc2x14_400_user_data_q1/1 -> conv3/1(In1)
  conv3/1(Out1) -> data_q1/1

== system xps_library/ADCs/adc2x14_400_4x ==
  conv : Subsystem
      mask help:
      | Converts an (14-bit) unsigned number to 2's complement.
      | This block should eventually be able to handle arbitrary
      | width inputs.
  conv1 : Subsystem
      mask help:
      | Converts an (14-bit) unsigned number to 2's complement.
      | This block should eventually be able to handle arbitrary
      | width inputs.
  conv2 : Subsystem
      mask help:
      | Converts an (14-bit) unsigned number to 2's complement.
      | This block should eventually be able to handle arbitrary
      | width inputs.
  conv3 : Subsystem
      mask help:
      | Converts an (14-bit) unsigned number to 2's complement.
      | This block should eventually be able to handle arbitrary
      | width inputs.
  conv4 : Subsystem
      mask help:
      | Converts an (14-bit) unsigned number to 2's complement.
      | This block should eventually be able to handle arbitrary
      | width inputs.
  conv5 : Subsystem
      mask help:
      | Converts an (14-bit) unsigned number to 2's complement.
      | This block should eventually be able to handle arbitrary
      | width inputs.
  conv6 : Subsystem
      mask help:
      | Converts an (14-bit) unsigned number to 2's complement.
      | This block should eventually be able to handle arbitrary
      | width inputs.
  conv7 : Subsystem
      mask help:
      | Converts an (14-bit) unsigned number to 2's complement.
      | This block should eventually be able to handle arbitrary
      | width inputs.
  xps_library_ADCs_adc2x14_400_4x_user_data_i{0..3} (4 alike) : xbsIndex_r4/Gateway In  gui_display_data_type=Fixed-point  arith_type=Unsigned  n_bits=14  bin_pt=0  preci_type=Single  exp_width=8  frac_width=24  quantization=Truncate  overflow=Wrap  period=1  dbl_ovrd=off  timing_constraint=None  locs_specified=off  LOCs={}  hdl_port=on  block_type=gatewayin
      settings: infoedit="Gateway in block.  Converts inputs of type Simulink integer, double and fixed point to  Xilinx fixed point type.<P><P>Hardware notes:  In hardware these blocks become top level input ports."  xl_area=[0, 0, 0, 0, 0, 0, 0]  block_version=10.1.3
  xps_library_ADCs_adc2x14_400_4x_user_data_q{0..3} (4 alike) : xbsIndex_r4/Gateway In  gui_display_data_type=Fixed-point  arith_type=Unsigned  n_bits=14  bin_pt=0  preci_type=Single  exp_width=8  frac_width=24  quantization=Truncate  overflow=Wrap  period=1  dbl_ovrd=off  timing_constraint=None  locs_specified=off  LOCs={}  hdl_port=on  block_type=gatewayin
      settings: infoedit="Gateway in block.  Converts inputs of type Simulink integer, double and fixed point to  Xilinx fixed point type.<P><P>Hardware notes:  In hardware these blocks become top level input ports."  xl_area=[0, 0, 0, 0, 0, 0, 0]  block_version=10.1.3
  xps_library_ADCs_adc2x14_400_4x_user_sync : xbsIndex_r4/Gateway In  gui_display_data_type=Fixed-point  arith_type=Boolean  n_bits=1  bin_pt=0  preci_type=Single  exp_width=8  frac_width=24  quantization=Truncate  overflow=Wrap  period=1  dbl_ovrd=off  timing_constraint=None  locs_specified=off  LOCs={}  hdl_port=on  block_type=gatewayin
      settings: infoedit="Gateway in block.  Converts inputs of type Simulink integer, double and fixed point to  Xilinx fixed point type.<P><P>Hardware notes:  In hardware these blocks become top level input ports."  xl_area=[0, 0, 0, 0, 0, 0, 0]  block_version=10.1.3
  data_i0 : Outport
  data_i1 : Outport  Port=2
  data_i2 : Outport  Port=3
  data_i3 : Outport  Port=4
  data_q0 : Outport  Port=5
  data_q1 : Outport  Port=6
  data_q2 : Outport  Port=7
  data_q3 : Outport  Port=8
  sync : Outport  Port=9
  wires:
  conv5/1(Out1) -> data_q1/1
  xps_library_ADCs_adc2x14_400_4x_user_data_q1/1 -> conv5/1(In1)
  conv1/1(Out1) -> data_i1/1
  xps_library_ADCs_adc2x14_400_4x_user_data_i1/1 -> conv1/1(In1)
  conv4/1(Out1) -> data_q0/1
  xps_library_ADCs_adc2x14_400_4x_user_data_q0/1 -> conv4/1(In1)
  conv/1(Out1) -> data_i0/1
  xps_library_ADCs_adc2x14_400_4x_user_data_i0/1 -> conv/1(In1)
  xps_library_ADCs_adc2x14_400_4x_user_sync/1 -> sync/1
  conv2/1(Out1) -> data_i2/1
  xps_library_ADCs_adc2x14_400_4x_user_data_i2/1 -> conv2/1(In1)
  conv3/1(Out1) -> data_i3/1
  xps_library_ADCs_adc2x14_400_4x_user_data_i3/1 -> conv3/1(In1)
  conv6/1(Out1) -> data_q2/1
  xps_library_ADCs_adc2x14_400_4x_user_data_q2/1 -> conv6/1(In1)
  conv7/1(Out1) -> data_q3/1
  xps_library_ADCs_adc2x14_400_4x_user_data_q3/1 -> conv7/1(In1)
